simulink model "untitled"  (R2025b)
settings: Solver=ode1be  StartTime=0.0  StopTime=15  FixedStep=0.001  RelTol=1e-3
undefined symbols (not defined in the file): DiscIntNeverNeededParam, X, Y, Z
libraries: sm_lib x94, nesl_utility x30, fl_lib x14, ee_lib x5, simulink_extras x4, instrumentseriallib x4, etargetslib x3
(part 1 of 4)
settings Model: Creator=송성혁  LastModifiedBy=송성혁
settings OptimizationCC: DefaultParameterBehavior=Inlined  EnhancedBackFolding=on  PassReuseOutputArgsAs=Individual arguments  ZeroExternalMemoryAtStartup=off  ZeroInternalMemoryAtStartup=off  OptimizeBlockOrder=speed  DifferentSizesBufferReuse=on  OptimizationCustomize=off  EfficientTunableParamExpr=on
settings DebuggingCC: ParameterTunabilityLossMsg=error
settings HardwareCC: ProdBitPerPointer=32.0  ProdBitPerSizeT=32.0  ProdBitPerPtrDiffT=32.0  ProdLargestAtomicFloat=None  ProdWordSize=32.0  ProdHWDeviceType=Custom Processor->Custom Processor
settings SFSimCC: MATLABDynamicMemAlloc=off
settings RTWCC: SystemTargetFile=ert.tlc  GenCodeOnly=on  TemplateMakefile=ert_default_tmf  Description=Embedded Coder
settings CodeAppCC: ForceParamTrailComments=on  IgnoreCustomStorageClasses=off  OperatorAnnotations=on  SimulinkDataObjDesc=on  SFDataObjDesc=on  InsertBlockDesc=on
settings ERTTargetCC: ERTCustomFileTemplate=example_file_process.tlc  TargetLangStandard=C99 (ISO)  GenerateSampleERTMain=on

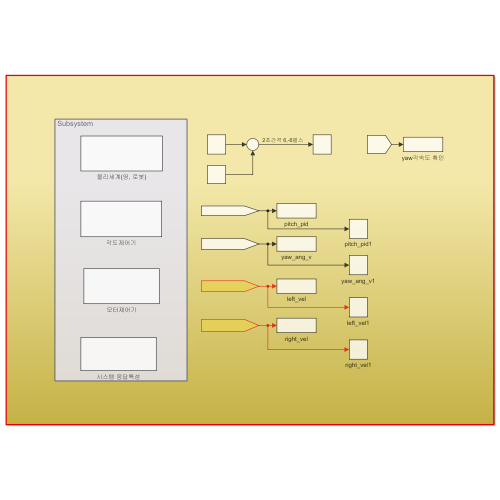
[thumbnail: Simulink's stored preview of the top-level diagram]
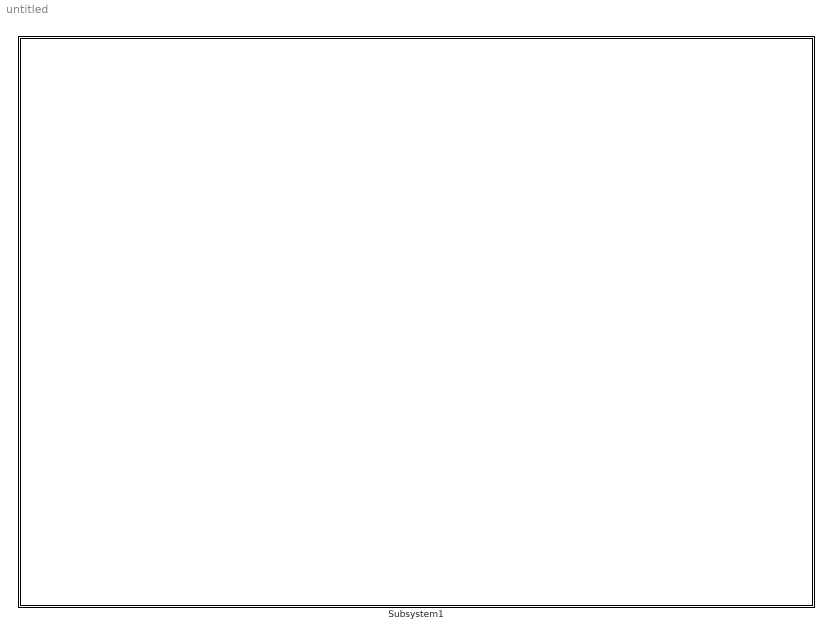
== system untitled ==
  Subsystem1 : Subsystem  TreatAsAtomicUnit=on

== system untitled/Subsystem1 ==
  note: Subsystem
  Constant1 : Constant  Value=-6
  Pulse Generator : DiscretePulseGenerator  PulseType=Time based  Amplitude=12  Period=4  PulseWidth=50
  Scope1 : Scope
      settings: ActiveDisplayYMinimum=-11.853878739880011  ActiveDisplayYMaximum=11.891103316870886  DataLoggingVariableName=ScopeData4
  Sum1 : Sum  Inputs=|++
  left_vel : Display
  left_vel1 : Scope
      settings: ActiveDisplayYMinimum=-0.33629965411154017  ActiveDisplayYMaximum=1.200157175202945  DataLoggingVariableName=ScopeData19
  pitch_pid : Display
  pitch_pid1 : Scope
      settings: DataLoggingVariableName=ScopeData16
  right_vel : Display
  right_vel1 : Scope
      settings: ActiveDisplayYMinimum=-1  ActiveDisplayYMaximum=1  DataLoggingVariableName=ScopeData20
  yaw_ang_v : Display
  yaw_ang_v1 : Scope
      settings: ActiveDisplayYMinimum=-1  ActiveDisplayYMaximum=1  DataLoggingVariableName=ScopeData18
  yaw각속도 확인 : Display
  각도제어기 : Subsystem
  모터제어기 : Subsystem
  "물리세계(땅, 로봇)" : Subsystem
  시스템 응답특성 : Subsystem
  wires:
  [yaw_ang_v] -> yaw_ang_v1/1, yaw_ang_v/1
  Constant1/1 -> Sum1/2
  [pitch_pid] -> pitch_pid1/1, pitch_pid/1
  [pitch] -> yaw각속도 확인/1
  Pulse Generator/1 -> Sum1/1
  Sum1/1 -> Scope1/1  "2초간격 6,-6펄스"
  [left_vel] -> left_vel1/1, left_vel/1
  [right_vel] -> right_vel1/1, right_vel/1

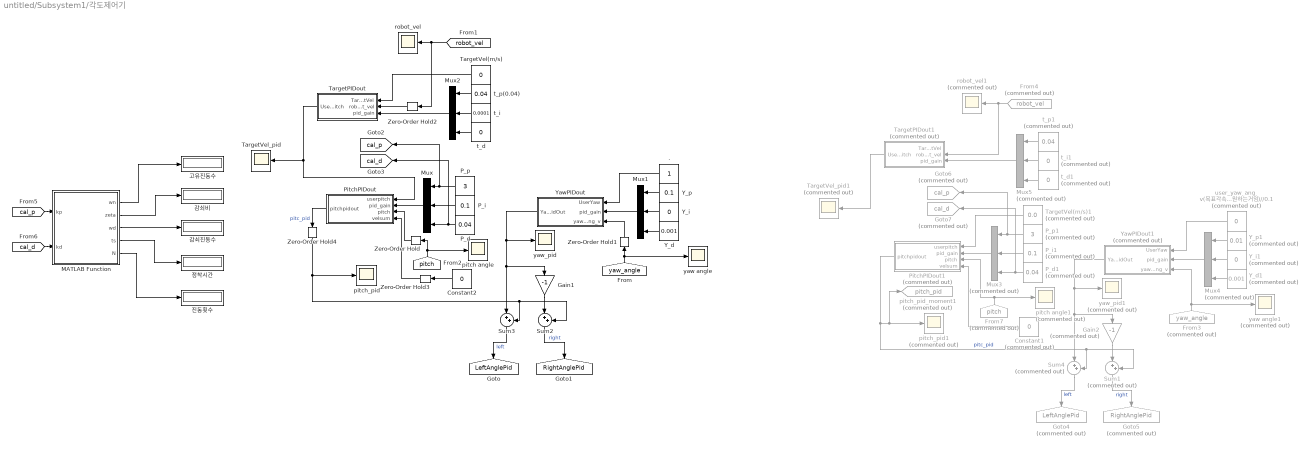
== system untitled/Subsystem1/각도제어기 ==
  . : Constant
  Constant1 : Constant  Commented=on  Value=0
  Constant2 : Constant  Value=0
  From3 : From  Commented=on  GotoTag=yaw_angle  TagVisibility=global
  From4 : From  Commented=on  GotoTag=robot_vel  TagVisibility=global
  From7 : From  Commented=on  GotoTag=pitch  TagVisibility=global
  Gain1 : Gain  Gain=-1
  Gain2 : Gain  Commented=on  Gain=-1
  Goto4 : Goto  Commented=on  GotoTag=LeftAnglePid  TagVisibility=global
  Goto5 : Goto  Commented=on  GotoTag=RightAnglePid  TagVisibility=global
  Goto6 : Goto  Commented=on  GotoTag=cal_p  TagVisibility=global
  Goto7 : Goto  Commented=on  GotoTag=cal_d  TagVisibility=global
  MATLAB Function : MATLAB Function  TreatAsAtomicUnit=on
  Mux : Mux  Inputs=3
  Mux1 : Mux  Inputs=3
  Mux2 : Mux  Inputs=3
  Mux3 : Mux  Commented=on  Inputs=3
  Mux4 : Mux  Commented=on  Inputs=3
  Mux5 : Mux  Commented=on  Inputs=3
  P_d : Constant  Value=0.04
  P_d1 : Constant  Commented=on  Value=0.04
  P_i : Constant  Value=0.1
  P_i1 : Constant  Commented=on  Value=0.1
  P_p : Constant  Value=3
  P_p1 : Constant  Commented=on  Value=3
  PitchPIDout : Subsystem
  PitchPIDout1 : Subsystem  Commented=on
  Sum1 : Sum  Commented=on  Inputs=|++
  Sum2 : Sum  Inputs=|++
  Sum3 : Sum  Inputs=|++
  Sum4 : Sum  Commented=on  Inputs=|++
  TargetPIDout : Subsystem
  TargetPIDout1 : Subsystem  Commented=on
  TargetVel(m/s) : Constant  Value=0
  TargetVel(m/s)1 : Constant  Commented=on  Value=0.0
  TargetVel_pid : Scope
      settings: ActiveDisplayYMinimum=0.0079999999998989768  ActiveDisplayYMaximum=0.00800000000090922  DataLoggingVariableName=ScopeData27
  TargetVel_pid1 : Scope  Commented=on
      settings: ActiveDisplayYMinimum=-0.00092878326566240372  ActiveDisplayYMaximum=0.0088888493334678739  DataLoggingVariableName=ScopeData37
  Y_d : Constant  Value=0.001
  Y_d1 : Constant  Commented=on  Value=0.001
  Y_i : Constant  Value=0
  Y_i1 : Constant  Commented=on  Value=0
  Y_p : Constant  Value=0.1
  Y_p1 : Constant  Commented=on  Value=0.01
  YawPIDout : Subsystem
  YawPIDout1 : Subsystem  Commented=on
  Zero-Order Hold{,1..4} (5 alike) : ZeroOrderHold  SampleTime=0.005
  pitch angle : Scope
      settings: ActiveDisplayYMinimum=-1  ActiveDisplayYMaximum=1  DataLoggingVariableName=ScopeData6
  pitch angle1 : Scope  Commented=on
      settings: ActiveDisplayYMinimum=-4.8560368908895039E-5  ActiveDisplayYMaximum=0.00043704332018005106  DataLoggingVariableName=ScopeData38
  pitch_pid : Scope
      settings: ActiveDisplayYMinimum=-0.034531364435790246  ActiveDisplayYMaximum=0.046434973047575975
  pitch_pid1 : Scope  Commented=on
      settings: ActiveDisplayYMinimum=-0.034531364435790246  ActiveDisplayYMaximum=0.046434973047575975  DataLoggingVariableName=ScopeData39
  pitch_pid_moment1 : Goto  Commented=on  GotoTag=pitch_pid  TagVisibility=global
  robot_vel : Scope
      settings: ActiveDisplayYMinimum=-0.17908515591336396  ActiveDisplayYMaximum=0.24602714480009077  DataLoggingVariableName=ScopeData24
  robot_vel1 : Scope  Commented=on
      settings: ActiveDisplayYMinimum=-0.4079570203605809  ActiveDisplayYMaximum=0.19738826011255114  DataLoggingVariableName=ScopeData40
  t_d : Constant  Value=0
  t_d1 : Constant  Commented=on  Value=0
  t_i : Constant  Value=0.0001
  t_i1 : Constant  Commented=on  Value=0
  t_p(0.04) : Constant  Value=0.04
  t_p1 : Constant  Commented=on  Value=0.04
  user_yaw_ang_v(목표각속도가 -이면 시계방향회전을 원하는거임)//0.1 : Constant  Commented=on  Value=0
  yaw angle : Scope
      settings: ActiveDisplayYMinimum=-3.9262838688053541  ActiveDisplayYMaximum=3.9268959912863686  DataLoggingVariableName=ScopeData11
  yaw angle1 : Scope  Commented=on
      settings: ActiveDisplayYMinimum=-3.9262838688053541  ActiveDisplayYMaximum=3.9268959912863686  DataLoggingVariableName=ScopeData41
  yaw_pid : Scope
      settings: ActiveDisplayYMinimum=-0.039201273453773333  ActiveDisplayYMaximum=0.10260469008728454  DataLoggingVariableName=ScopeData21
  yaw_pid1 : Scope  Commented=on
      settings: ActiveDisplayYMinimum=-0.039201273453773333  ActiveDisplayYMaximum=0.10260469008728454  DataLoggingVariableName=ScopeData42
  감쇠비 : Display
  감쇠진동수 : Display
  고유진동수 : Display
  정착시간 : Display
  진동횟수 : Display
  tag scope: LeftAnglePid=global, RightAnglePid=global, cal_d=global, cal_p=global
  wires:
  Y_d/1 -> Mux1/3
  P_i/1 -> Mux/2
  PitchPIDout/1(pitchpidout) -> Zero-Order Hold4/1  "pitc_pid"
  Y_p/1 -> Mux1/1
  P_p/1 -> [cal_p], Mux/1
  Sum2/1 -> [RightAnglePid]  "right"
  Y_i/1 -> Mux1/2
  Sum3/1 -> [LeftAnglePid]  "left"
  Mux/1 -> PitchPIDout/2(pid_gain)
  ./1 -> YawPIDout/1(UserYaw)
  Mux1/1 -> YawPIDout/2(pid_gain)
  YawPIDout/1(YawPidOut) -> Gain1/1, Sum3/1, yaw_pid/1
  Gain1/1 -> Sum2/1
  [pitch] -> Zero-Order Hold/1, pitch angle/1
  [yaw_angle] -> yaw angle/1, Zero-Order Hold1/1
  P_d/1 -> [cal_d], Mux/3
  t_i/1 -> Mux2/2
  t_d/1 -> Mux2/3
  Mux2/1 -> TargetPIDout/3(pid_gain)
  t_p(0.04)/1 -> Mux2/1
  [robot_vel] -> Zero-Order Hold2/1, robot_vel/1
  MATLAB Function/2(zeta) -> 감쇠비/1
  MATLAB Function/4(ts) -> 정착시간/1
  MATLAB Function/1(wn) -> 고유진동수/1
  MATLAB Function/3(wd) -> 감쇠진동수/1
  [cal_p] -> MATLAB Function/1(kp)
  [cal_d] -> MATLAB Function/2(kd)
  MATLAB Function/5(N) -> 진동횟수/1
  Zero-Order Hold/1 -> PitchPIDout/3(pitch)
  Zero-Order Hold1/1 -> YawPIDout/3(yaw_ang_v)
  Zero-Order Hold2/1 -> TargetPIDout/2(robot_vel)
  Constant2/1 -> Zero-Order Hold3/1
  Zero-Order Hold3/1 -> PitchPIDout/4(velsum)
  Zero-Order Hold4/1 -> pitch_pid/1, Sum3/2, Sum2/2
  PitchPIDout1/1(pitchpidout) -> pitch_pid_moment1/1, pitch_pid1/1, Sum4/2, Sum1/2  "pitc_pid"
  From3/1 -> YawPIDout1/3(yaw_ang_v), yaw angle1/1
  Constant1/1 -> PitchPIDout1/4(velsum)
  YawPIDout1/1(YawPidOut) -> Gain2/1, Sum4/1, yaw_pid1/1
  Mux3/1 -> PitchPIDout1/2(pid_gain)
  Gain2/1 -> Sum1/1
  Sum1/1 -> Goto5/1  "right"
  Y_i1/1 -> Mux4/2
  P_d1/1 -> Goto7/1, Mux3/3
  user_yaw_ang_v(목표각속도가 -이면 시계방향회전을 원하는거임)//0.1/1 -> YawPIDout1/1(UserYaw)
  Sum4/1 -> Goto4/1  "left"
  From7/1 -> PitchPIDout1/3(pitch), pitch angle1/1
  Y_d1/1 -> Mux4/3
  t_p1/1 -> Mux5/1
  From4/1 -> TargetPIDout1/2(robot_vel), robot_vel1/1
  Mux4/1 -> YawPIDout1/2(pid_gain)
  P_i1/1 -> Mux3/2
  Mux5/1 -> TargetPIDout1/3(pid_gain)
  t_d1/1 -> Mux5/3
  TargetPIDout1/1(UserPitch) -> TargetVel_pid1/1
  TargetVel(m/s)1/1 -> PitchPIDout1/1(userpitch)
  P_p1/1 -> Goto6/1, Mux3/1
  t_i1/1 -> Mux5/2
  Y_p1/1 -> Mux4/1
  TargetPIDout/1(UserPitch) -> PitchPIDout/1(userpitch), TargetVel_pid/1
  TargetVel(m/s)/1 -> TargetPIDout/1(TargetVel)

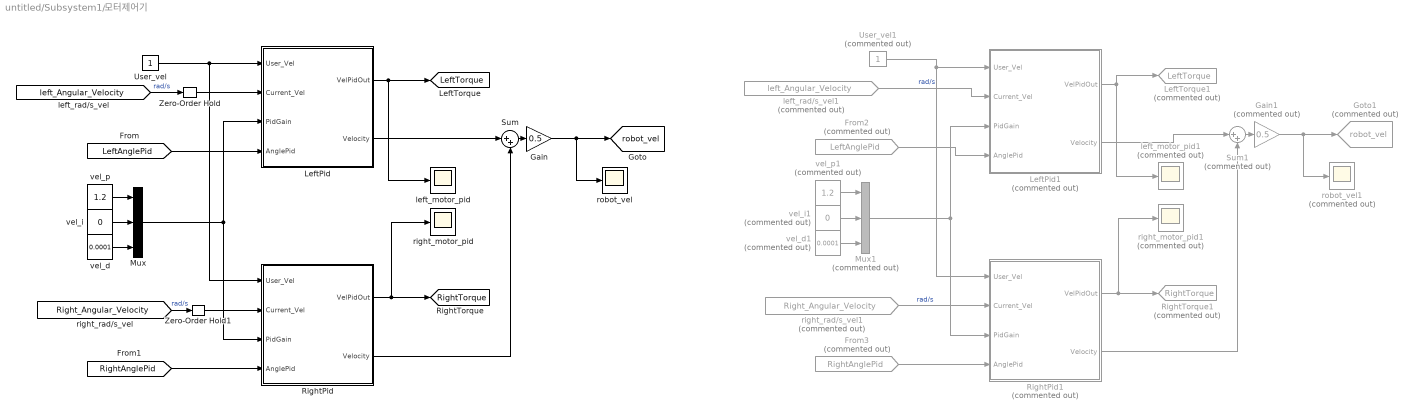
== system untitled/Subsystem1/모터제어기 ==
  From2 : From  Commented=on  GotoTag=LeftAnglePid  TagVisibility=global
  From3 : From  Commented=on  GotoTag=RightAnglePid  TagVisibility=global
  Gain : Gain  Gain=0.5
  Gain1 : Gain  Commented=on  Gain=0.5
  Goto1 : Goto  Commented=on  GotoTag=robot_vel  TagVisibility=global
  LeftPid : Subsystem
  LeftPid1 : Subsystem  Commented=on
  LeftTorque1 : Goto  Commented=on  GotoTag=LeftTorque  TagVisibility=global
  Mux : Mux  Inputs=3
  Mux1 : Mux  Commented=on  Inputs=3
  RightPid : Subsystem
  RightPid1 : Subsystem  Commented=on
  RightTorque1 : Goto  Commented=on  GotoTag=RightTorque  TagVisibility=global
  Sum : Sum  Inputs=|++
  Sum1 : Sum  Commented=on  Inputs=|++
  User_vel : Constant
  User_vel1 : Constant  Commented=on
  Zero-Order Hold : ZeroOrderHold  SampleTime=0.005
  Zero-Order Hold1 : ZeroOrderHold  SampleTime=0.005
  left_motor_pid : Scope
      settings: ActiveDisplayYMinimum=-0.029471180633000547  ActiveDisplayYMaximum=0.024626331118496228  DataLoggingVariableName=ScopeData12
  left_motor_pid1 : Scope  Commented=on
      settings: ActiveDisplayYMinimum=-0.029471180633000547  ActiveDisplayYMaximum=0.024626331118496228  DataLoggingVariableName=ScopeData43
  left_rad/s_vel1 : From  Commented=on  GotoTag=left_Angular_Velocity  TagVisibility=global
  right_motor_pid : Scope
      settings: ActiveDisplayYMinimum=-0.03418278216021374  ActiveDisplayYMaximum=0.05052958775636103  DataLoggingVariableName=ScopeData10
  right_motor_pid1 : Scope  Commented=on
      settings: ActiveDisplayYMinimum=-0.03418278216021374  ActiveDisplayYMaximum=0.05052958775636103  DataLoggingVariableName=ScopeData44
  right_rad/s_vel1 : From  Commented=on  GotoTag=Right_Angular_Velocity  TagVisibility=global
  robot_vel : Scope
      settings: ActiveDisplayYMinimum=-0.9251081456236363  ActiveDisplayYMaximum=3.3137002553325159  DataLoggingVariableName=ScopeData26
  robot_vel1 : Scope  Commented=on
      settings: ActiveDisplayYMinimum=-0.9251081456236363  ActiveDisplayYMaximum=3.3137002553325159  DataLoggingVariableName=ScopeData45
  vel_d : Constant  Value=0.0001
  vel_d1 : Constant  Commented=on  Value=0.0001
  vel_i : Constant  Value=0
  vel_i1 : Constant  Commented=on  Value=0
  vel_p : Constant  Value=1.2
  vel_p1 : Constant  Commented=on  Value=1.2
  tag scope: LeftTorque=global, RightTorque=global, robot_vel=global
  wires:
  User_vel/1 -> RightPid/1(User_Vel), LeftPid/1(User_Vel)
  Mux/1 -> RightPid/3(PidGain), LeftPid/3(PidGain)
  [LeftAnglePid] -> LeftPid/4(AnglePid)
  [RightAnglePid] -> RightPid/4(AnglePid)
  vel_p/1 -> Mux/1
  vel_i/1 -> Mux/2
  vel_d/1 -> Mux/3
  RightPid/1(VelPidOut) -> [RightTorque], right_motor_pid/1
  LeftPid/1(VelPidOut) -> [LeftTorque], left_motor_pid/1
  LeftPid/2(Velocity) -> Sum/1
  RightPid/2(Velocity) -> Sum/2
  Sum/1 -> Gain/1
  Gain/1 -> robot_vel/1, [robot_vel]
  [left_Angular_Velocity] -> Zero-Order Hold/1  "rad/s"
  Zero-Order Hold/1 -> LeftPid/2(Current_Vel)
  [Right_Angular_Velocity] -> Zero-Order Hold1/1  "rad/s"
  Zero-Order Hold1/1 -> RightPid/2(Current_Vel)
  Gain1/1 -> robot_vel1/1, Goto1/1
  LeftPid1/2(Velocity) -> Sum1/1
  vel_p1/1 -> Mux1/1
  right_rad/s_vel1/1 -> RightPid1/2(Current_Vel)  "rad/s"
  vel_d1/1 -> Mux1/3
  left_rad/s_vel1/1 -> LeftPid1/2(Current_Vel)  "rad/s"
  Mux1/1 -> RightPid1/3(PidGain), LeftPid1/3(PidGain)
  vel_i1/1 -> Mux1/2
  From2/1 -> LeftPid1/4(AnglePid)
  Sum1/1 -> Gain1/1
  User_vel1/1 -> RightPid1/1(User_Vel), LeftPid1/1(User_Vel)
  RightPid1/1(VelPidOut) -> RightTorque1/1, right_motor_pid1/1
  From3/1 -> RightPid1/4(AnglePid)
  RightPid1/2(Velocity) -> Sum1/2
  LeftPid1/1(VelPidOut) -> LeftTorque1/1, left_motor_pid1/1
